simulink model "NEPTUN_ZH_Z2"  (R2026a)
settings: Solver=VariableStepAuto  StopTime=25  MaxStep=100e-3
libraries: simulink_extras x1
settings Model: Creator=Szalay  LastModifiedBy=Szalay

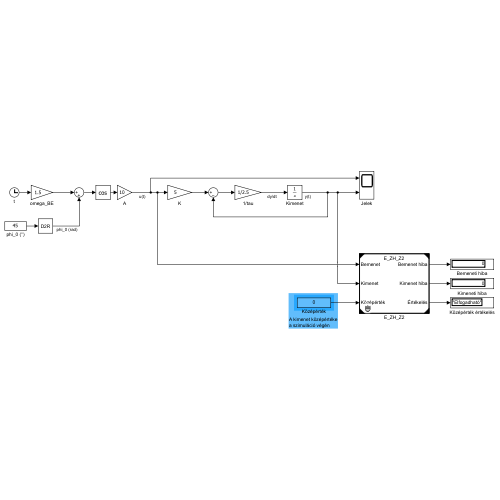
[thumbnail: Simulink's stored preview of the top-level diagram]
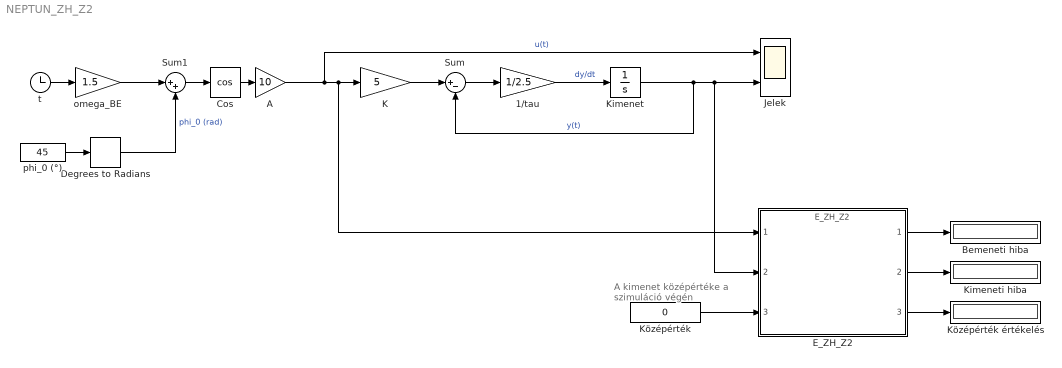
== system NEPTUN_ZH_Z2 ==
  note: A kimenet középértéke
      | a szimuláció végén
  1/tau : Gain  Gain=1/2.5
  A : Gain  Gain=10
  Bemeneti hiba : Display
  Cos : Trigonometry  Operator=cos
  Degrees to Radians : simulink_extras/Transformations/Degrees to Radians
  E_ZH_Z2 : ModelReference  ModelNameDialog=E_ZH_Z2.slxp  ModelReferenceVersion=3.3  CopyOfModelProtected=on
  Jelek : Scope  NumInputPorts=2
      settings: ActiveDisplayYMinimum=-12.497130037104094  ActiveDisplayYMaximum=12.498636325994815
  K : Gain  Gain=5
  Kimenet : Integrator  InitialCondition=-20
  Kimeneti hiba : Display
  Középérték : Constant  Value=0
  Középérték értékelés : Display
  Sum : Sum  Inputs=|+-
  Sum1 : Sum  Inputs=|++
  omega_BE : Gain  Gain=1.5
  phi_0 (°) : Constant  Value=45
  t : Clock
  wires:
  E_ZH_Z2/1 -> Bemeneti hiba/1
  E_ZH_Z2/2 -> Kimeneti hiba/1
  E_ZH_Z2/3 -> Középérték értékelés/1
  Középérték/1 -> E_ZH_Z2/3
  Kimenet/1 -> Sum/2, E_ZH_Z2/2, Jelek/2  "y(t)"
  1/tau/1 -> Kimenet/1  "dy/dt"
  Sum/1 -> 1/tau/1
  K/1 -> Sum/1
  A/1 -> Jelek/1, E_ZH_Z2/1, K/1  "u(t)"
  Cos/1 -> A/1
  Sum1/1 -> Cos/1
  omega_BE/1 -> Sum1/1
  t/1 -> omega_BE/1
  phi_0 (°)/1 -> Degrees to Radians/1
  Degrees to Radians/1 -> Sum1/2  "phi_0 (rad)"
